simulink subsystem "Subsys_GFolConv_Control"  (R2024b)
settings: Solver=VariableStepAuto  StartTime=0.0  StopTime=10.0  RelTol=1e-3
model mask{S_n=2e6, P_binst=1.5e6, f_n=50, V_n_phph=690, V_n_grid_phph=20e3, V_n_dc=1380, L_filter_conv_pu=[ 0.0001 0.05097 ], C_filter_pu=[ 0.06875 0.04569 ], outputSignal=0, f_sw=5000, send_info_messages=1, T_s_ctrl=1e-4, T_s_PWM_meas=1e-4, datatype='double', meas_signals=0, meas_lowpass=1, meas_f_cutoff_lowpass=2500, meas_f_cutoff_posseq=20, prot_variant=2, v_dc_max=1.2, v_ac_max=1.1, t_ac_max=0.1, v_ac_maxmax=1.25, t_ac_maxmax=0.1, v_ac_min=0.8, t_ac_min=3, v_ac_minmin=0.45, t_ac_minmin=0.3, f_ac_max=51.5, t_f_ac_max=0.1, f_ac_maxmax=52.5, t_f_ac_maxmax=10, f_ac_min=47.5, t_f_ac_min=0.1, i_ac_max=1.25, outer_ctrl_mode=1, VDE4110_T_LPF_P=33e-3, VDE4110_Pf_DBlow=49.8, VDE4110_Pf_DBhigh=50.2, VDE4110_Pf_droop=5, VDE4110_Pf_dPdtmax=1, isStorage=0, Ts_Matching_m=0, K_Matching_m=0, Plant_Ref=0, Plant_Model=0, Luenberger=0, VDE4110_Q_ctrl_mode=3, VDE4110_T_PT1_Q=3.33, VDE4110_QV_uq0ref=1, VDE4110_QV_qmax=0.33, VDE4110_QV_umax=1.04, VDE4110_QV_deadband=0, VDE4110_QP_P=[0.1, 0.5, 0.6, 0.9, 1.0], VDE4110_QP_Q=[0.0, 0.0, -0.05, -0.33, -0.33], VDE4110_QVDB_P1=[0.94, 0.33], VDE4110_QVDB_P2=[0.96, 0], VDE4110_QVDB_P3=[1.04, 0], VDE4110_QVDB_P4=[1.06, -0.33], VDE4110_cosphi_ref=1, VDE4110_cosphi_direction=1, PQ_ctrl_mode=0, K_p_PQ_Ctrl=0.6, K_i_PQ_Ctrl=3.2, K_p_I_Ctrl=0.6, K_i_I_Ctrl=0.6, v_conv_max=1.3, i_grid_max=1.1, active_damping=1, R_virt_pu=0.2}
  mask prompts: S_n "Nominal apparent power [VA]"; P_binst "Installed active power [W]"; f_n "Nominal frequency [Hz]"; V_n_phph "Nominal converter voltage (rms, phase-to-phase) [V]"; V_n_grid_phph "Nominal grid voltage (rms, phase-to-phase) [V]"; V_n_dc "Nominal DC-link voltage [V]"; L_filter_conv_pu "Impedance of converter-side inductance [ R L ] (pu)"; C_filter_pu "Impedance of filter capacitor [ R C ] (pu)"; outputSignal "Output signal type (2 = duty cycle (imperix), 1 = switching pulses, 0 = voltage reference (average model))"; f_sw "Switching frequency [Hz]"; send_info_messages "Send info messages (1 = enabled, 0 = disabled)"; T_s_ctrl "Controller sample time [s]"; T_s_PWM_meas "PWM and measurements sample time [s]"; datatype "Signal data type"; meas_signals "Measured signals (0 = all signals (tDMSquared simulation), 1 = reduced signals (imperix hardware))"; meas_lowpass "Low pass to filter measurement noise (1 = enabled, 0 = disabled)"; meas_f_cutoff_lowpass "Cutoff frequency of low pass filter (measurement noise) [Hz]"; meas_f_cutoff_posseq "Cutoff frequency of low pass filter (positive sequence calculation) [Hz]"; prot_variant "Protection Variant (1= hardware protection, 2 = tDMSquared warnings only, 3 = deactivated)"; v_dc_max "Maximum DC-link voltage [% nom. value]"; v_ac_max "Lower Maximum AC voltage [% nom. value]"; t_ac_max "Lower Maximum AC voltage timing [s]"; v_ac_maxmax "Upper Maximum AC voltage [% nom. value]"; t_ac_maxmax "Upper Maximum AC voltage timing [s]"; v_ac_min "Upper Minimum AC voltage [% nom. value]"; t_ac_min "Upper Minimum AC voltage timing [s]"; v_ac_minmin "Lower Minimum AC voltage [% nom. value]"; t_ac_minmin "Lower Minimum AC voltage timing [s]"; f_ac_max "Maximum AC frequency [Hz]"; t_f_ac_max "Maximum AC frequency timing [s]"; f_ac_maxmax "Upper Maximum AC frequency [Hz]"; t_f_ac_maxmax "Upper Maximum AC frequency timing [s]"; f_ac_min "Minimum AC frequency [Hz]"; t_f_ac_min "Minimum AC frequency timing [s]"; i_ac_max "Maximum AC current [% nom. value]"; outer_ctrl_mode "Outer control mode (1 = VDE 4110, 2 = Matching Control, 3 = no control)"; VDE4110_T_LPF_P "Time constant of active power  PT1 [s]"; VDE4110_Pf_DBlow "P(f) deadband lower limit [Hz]"; VDE4110_Pf_DBhigh "P(f) deadband higher limit [Hz]"; VDE4110_Pf_droop "P(f) droop [(df/f_n)/(dP/Pref)] [%]"; VDE4110_Pf_dPdtmax "P(f) maximum dP/dt [pu / s]"; isStorage "Generation unit is energy storage (1 = true, 0 = false)"; Ts_Matching_m "Time Constant"; K_Matching_m "Feedback Gain"; Plant_Ref "Reference Model"; Plant_Model "Plant Model"; Luenberger "Luenberger Gain"; VDE4110_Q_ctrl_mode "Q-control mode (1 = Q(V), 2 = Q(P), 3 = Q(V) with deadband, 4 = cosphi)"; VDE4110_T_PT1_Q "Time constant of reactive power PT1 delay [s]"; VDE4110_QV_uq0ref "U_Q0ref [pu]"; VDE4110_QV_qmax "|Q_max| [pu]"; VDE4110_QV_umax "U_max [pu]"; VDE4110_QV_deadband "Voltage deadband [+- %]"; VDE4110_QP_P "P_grid points [pu]"; VDE4110_QP_Q "Q_grid points [pu]"; VDE4110_QVDB_P1 "P1 [V_grid, Q_grid] [pu]"; VDE4110_QVDB_P2 "P2 [V_grid, Q_grid] [pu]"; VDE4110_QVDB_P3 "P3 [V_grid, Q_grid] [pu]"; VDE4110_QVDB_P4 "P4 [V_grid, Q_grid] [pu]"; VDE4110_cosphi_ref "cos(phi)"; VDE4110_cosphi_direction "Reactive power flow direction (1 = ind. Q injection, 0 = ind. Q consumption)"; PQ_ctrl_mode "Active/reactive power control mode (closed loop = 0, open loop = 1)"; K_p_PQ_Ctrl "Proportional gain (PI power controller) [pu]"; K_i_PQ_Ctrl "Integral gain (PI power controller) [pu]"; K_p_I_Ctrl "Proportional gain (PI current controller) [pu]"; K_i_I_Ctrl "Integral gain (PI current controller) [pu]"; v_conv_max "Converter voltage maximum value (limit) [pu]"; i_grid_max "Converter current maximum value (limit) [pu]"; active_damping "Active Damping (1 = enabled, 0 = disabled)"; R_virt_pu "Virtual resistor for active damping (in series with converter-side inductance) [pu]"
libraries: simulink x6, eeTransforms x2, eePwmGeneratorTwoLevel x1
settings Model: Creator=winkens  LastModifiedBy=KIVANÇKOCAOĞULLAR
settings SolverCC: AlgebraicLoopSolver=TrustRegion
settings OptimizationCC: ReuseModelBlockBuffer=off
settings DebuggingCC: UnconnectedInputMsg=warning  UnconnectedOutputMsg=warning  UnconnectedLineMsg=warning
settings ModelReferenceCC: EnableRefExpFcnMdlSchedulingChecks=on
settings RTWCC: GPUComputeCapability=3.5  DLArmComputeVersion=19.05

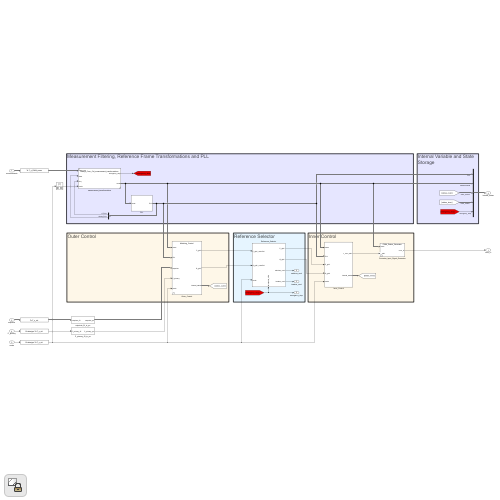
[thumbnail: Simulink's stored preview of the top-level diagram]
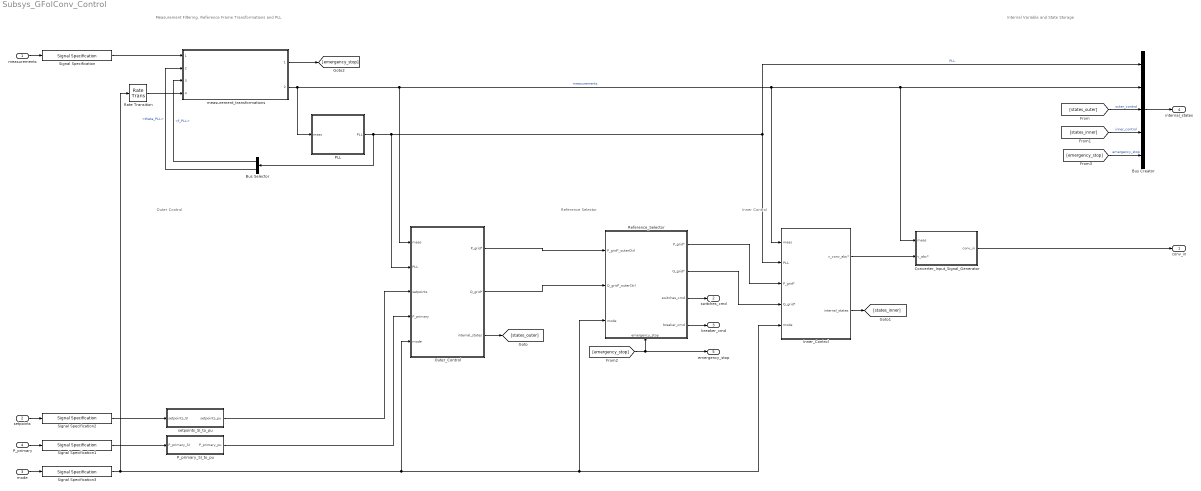
== system Subsys_GFolConv_Control ==
  note: Reference Selector
  note: Measurement Filtering, Reference Frame Transformations and PLL
  note: Outer Control
  note: Inner Control
  note: Internal Variable and State
      | Storage
  measurements : Inport
  setpoints : Inport  Port=2
  mode : Inport  Port=3
  P_primary : Inport  Port=4
  Bus Creator : BusCreator  Inputs=5
  Bus Selector : BusSelector  OutputSignals=f_PLL,theta_PLL
  Converter_Input_Signal_Generator : Subsystem  Variant=on
  Inner_Control : Subsystem
  Outer_Control : Subsystem  Variant=on  VariantControl=Choice
  PLL : Subsystem
  P_primary_SI_to_pu : Subsystem
  Rate Transition : RateTransition  OutPortSampleTime=T_s_PWM_meas
  Reference_Selector : Subsystem
      settings: PortSchema="{\"entries\":[{\"content\":{\"sides\":[{\"content\":{\"connectorIds\":[\"In1\",\"In2\",\"In3\"]},\"type\":\"ConnectorPlacement.EquallySpacedRectSide\",\"uuid\":\"b573c78f-d58c-40ce-b3bc-9375892f1426\"},{\"content\":{\"connectorIds\":[\"Out1\",\"Out2\",\"Out3\",\"Out4\"],\"side\":\"RIGHT\"},\"type\":\"ConnectorPlacement.EquallySpacedRectSide\",\"uuid\":\"e589ace7-4775-4159-9960-f42613345aac\"},{\"content\":{\"connectorIds\":[],\"side\":\"TOP\"},\"type\":\"ConnectorPlacement.EquallySpacedRectSide\",\"uuid\":\"d891a4af-dcc2-49f2-8d70-7d3294665827\"},{\"content\":{\"connectorIds\":[\"In4\"],\"side\":\"BOTTOM\"},\"type\":\"ConnectorPlacement.EquallySpacedRectSide\",\"uuid\":\"20ebcd43-a549-487f-8746-8af8878ad08b\"},{\"content\":{\"connectorIds\":[],\"side\":\"HIDDEN\"},\"type\":\"ConnectorPlacement.EquallySpacedRectSide\",\"uuid\":\"aa9de6de-879f-42fa-ad20-1b3327d10a74\"}]},\"type\":\"ConnectorPlacement.EquallySpacedConnector\",\"uuid\":\"970e3a91-45bd-4cb1-a5f8-11fb4fe15b0f\"}],\"packageUris\":[\"http://schema.mathworks.com/mf0/Connector/R2020b\"],\"version\":\"1.0\"}"
  Signal Specification : SignalSpecification  SampleTime=T_s_PWM_meas
  Signal Specification1 : SignalSpecification  OutDataTypeStr=datatype  SampleTime=T_s_ctrl
  Signal Specification2 : SignalSpecification  SampleTime=T_s_ctrl
  Signal Specification3 : SignalSpecification  OutDataTypeStr=datatype  SampleTime=T_s_ctrl
  measurement_transformations : Subsystem  ReferencedSubsystem=Subsys_Conv_Ctrl_measurement_transformations  S_n=S_n  f_n=f_n  V_n_phph=V_n_phph  V_n_grid_phph=V_n_grid_phph  V_n_dc=V_n_dc  meas_signals=meas_signals  meas_noise_filter=meas_lowpass  f_cutoff_lowpass=meas_f_cutoff_lowpass  posseq_calc=0  f_cutoff_posseq=meas_f_cutoff_posseq  prot_variant=prot_variant  v_dc_max=v_dc_max  v_ac_max=v_ac_max  t_ac_max=t_ac_max  v_ac_maxmax=v_ac_maxmax  t_ac_maxmax=t_ac_maxmax  v_ac_min=v_ac_min  t_ac_min=t_ac_min  v_ac_minmin=v_ac_minmin  t_ac_minmin=t_ac_minmin  f_ac_max=f_ac_max  t_f_ac_max=t_f_ac_max  f_ac_maxmax=f_ac_maxmax  t_f_ac_maxmax=t_f_ac_maxmax  f_ac_min=f_ac_min  t_f_ac_min=t_f_ac_min  i_ac_max=i_ac_max  T_s_ctrl=T_s_ctrl  T_s_PWM_meas=T_s_PWM_meas  datatype=datatype
  setpoints_SI_to_pu : Subsystem
  conv_in : Outport
  switches_cmd : Outport  Port=2
  breaker_cmd : Outport  Port=3
  internal_states : Outport  Port=4
  emergency_stop : Outport  Port=5
  wires:
  Bus Selector/1 -> measurement_transformations/3  "<f_PLL>"
  Reference_Selector/2(Q_grid*) -> Inner_Control/4(Q_grid*)
  Reference_Selector/1(P_grid*) -> Inner_Control/3(P_grid*)
  [emergency_stop] -> Reference_Selector/4(emergency_stop), emergency_stop/1
  Reference_Selector/3(switches_cmd) -> switches_cmd/1
  Reference_Selector/4(breaker_cmd) -> breaker_cmd/1
  Signal Specification2/1 -> setpoints_SI_to_pu/1(setpoints_SI)
  measurement_transformations/1 -> [emergency_stop]
  Bus Selector/2 -> measurement_transformations/2  "<theta_PLL>"
  Signal Specification/1 -> measurement_transformations/1
  Signal Specification3/1 -> Reference_Selector/3(mode), Inner_Control/5(mode), Outer_Control/5(mode), Rate Transition/1
  Signal Specification1/1 -> P_primary_SI_to_pu/1(P_primary_SI)
  P_primary_SI_to_pu/1(P_primary_pu) -> Outer_Control/4(P_primary)
  P_primary/1 -> Signal Specification1/1
  Outer_Control/3(internal_states) -> [states_outer]
  Outer_Control/2(Q_grid*) -> Reference_Selector/2(Q_grid*_outerCtrl)
  Outer_Control/1(P_grid*) -> Reference_Selector/1(P_grid*_outerCtrl)
  setpoints_SI_to_pu/1(setpoints_pu) -> Outer_Control/3(setpoints)
  measurements/1 -> Signal Specification/1
  setpoints/1 -> Signal Specification2/1
  mode/1 -> Signal Specification3/1
  measurement_transformations/2 -> PLL/1(meas), Outer_Control/1(meas), Bus Creator/2, Converter_Input_Signal_Generator/1(meas), Inner_Control/1(meas)  "measurements"
  Inner_Control/1(v_conv_abc*) -> Converter_Input_Signal_Generator/2(v_abc*)
  Inner_Control/2(internal_states) -> [states_inner]
  [states_outer] -> Bus Creator/3  "outer_control"
  [states_inner] -> Bus Creator/4  "inner_control"
  Bus Creator/1 -> internal_states/1
  Converter_Input_Signal_Generator/1(conv_in) -> conv_in/1
  [emergency_stop] -> Bus Creator/5  "emergency_stop"
  Rate Transition/1 -> measurement_transformations/4
  PLL/1(PLL) -> Bus Selector/1, Bus Creator/1, Inner_Control/2(PLL), Outer_Control/2(PLL)  "PLL"

== system Subsys_GFolConv_Control/Converter_Input_Signal_Generator ==
  meas : Inport
  v_abc* : Inport  Port=2
  PWM_Pulses_Generator : Subsystem  VariantControl=outputSignal == 1
  Uref_Signal_Generator : Subsystem  VariantControl=(default)
  imperix_dutycycle_generator : Subsystem  VariantControl=outputSignal == 2
  conv_in : Outport

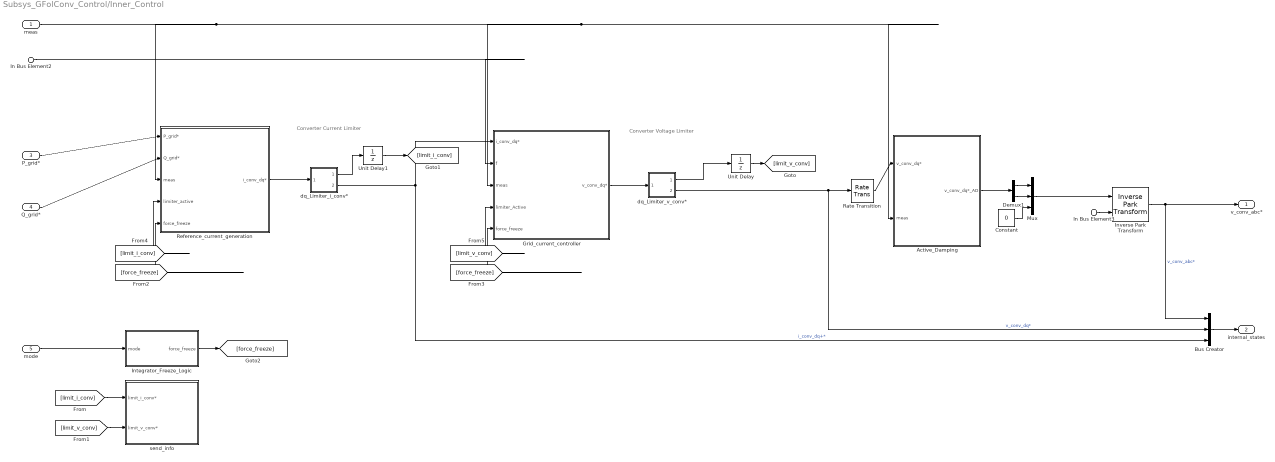
== system Subsys_GFolConv_Control/Inner_Control ==
  note: Converter Current Limiter
  note: Converter Voltage Limiter
  meas : Inport
  In Bus Element2 : Inport  Port=2  PortName=PLL  Element=f_PLL
  In Bus Element3 : Inport  Port=2  PortName=PLL  Element=theta_PLL
  P_grid* : Inport  Port=3
  Q_grid* : Inport  Port=4
  mode : Inport  Port=5
  Active_Damping : Subsystem  Variant=on  VariantControl=Choice
  Bus Creator : BusCreator  Inputs=3
  Constant : Constant  Value=0  OutDataTypeStr=datatype
  Demux1 : Demux  Outputs=2
  Grid_current_controller : Subsystem
  Integrator_Freeze_Logic : Subsystem
  Inverse Park Transform : eeTransforms/Inverse Park Transform  AxisAlignment=D-axis  PowerInvariant=off
  Mux : Mux  Inputs=3
  Rate Transition : RateTransition  Deterministic=off  OutPortSampleTime=T_s_PWM_meas
  Reference_current_generation : Subsystem  Variant=on  VariantControl=Choice
  Unit Delay : UnitDelay  SampleTime=-1  HasFrameUpgradeWarning=on
  Unit Delay1 : UnitDelay  SampleTime=-1  HasFrameUpgradeWarning=on
  dq_Limiter_i_conv* : Subsystem  ReferencedSubsystem=dq_Limiter  X_dq_max=i_grid_max  datatype=datatype
  dq_Limiter_v_conv* : Subsystem  ReferencedSubsystem=dq_Limiter  X_dq_max=v_conv_max  datatype=datatype
  send_info : Subsystem  Variant=on
  v_conv_abc* : Outport
  internal_states : Outport  Port=2
  wires:
  Integrator_Freeze_Logic/1(force_freeze) -> [force_freeze]
  mode/1 -> Integrator_Freeze_Logic/1(mode)
  Unit Delay1/1 -> [limit_i_conv]
  Reference_current_generation/1(i_conv_dq*) -> dq_Limiter_i_conv*/1
  dq_Limiter_i_conv*/1 -> Unit Delay1/1
  P_grid*/1 -> Reference_current_generation/1(P_grid*)
  Q_grid*/1 -> Reference_current_generation/2(Q_grid*)
  dq_Limiter_v_conv*/1 -> Unit Delay/1
  dq_Limiter_v_conv*/2 -> Bus Creator/2, Rate Transition/1  "v_conv_dq*"
  Unit Delay/1 -> [limit_v_conv]
  Mux/1 -> Inverse Park Transform/1
  Constant/1 -> Mux/3
  Demux1/2 -> Mux/2
  Demux1/1 -> Mux/1
  meas/1 -> Grid_current_controller/3(meas), Active_Damping/2(meas), Reference_current_generation/3(meas)
  In Bus Element2/1 -> Grid_current_controller/2(f)
  In Bus Element3/1 -> Inverse Park Transform/2
  Inverse Park Transform/1 -> Bus Creator/1, v_conv_abc*/1  "v_conv_abc*"
  Bus Creator/1 -> internal_states/1
  dq_Limiter_i_conv*/2 -> Bus Creator/3, Grid_current_controller/1(i_conv_dq*)  "i_conv_dq+*"
  Grid_current_controller/1(v_conv_dq*) -> dq_Limiter_v_conv*/1
  Rate Transition/1 -> Active_Damping/1(v_conv_dq*)
  Active_Damping/1(v_conv_dq*_AD) -> Demux1/1
  [limit_i_conv] -> send_info/1(limit_i_conv*)
  [limit_v_conv] -> send_info/2(limit_v_conv*)
  [force_freeze] -> Reference_current_generation/5(force_freeze)
  [force_freeze] -> Grid_current_controller/5(force_freeze)
  [limit_i_conv] -> Reference_current_generation/4(limiter_active)
  [limit_v_conv] -> Grid_current_controller/4(limiter_Active)

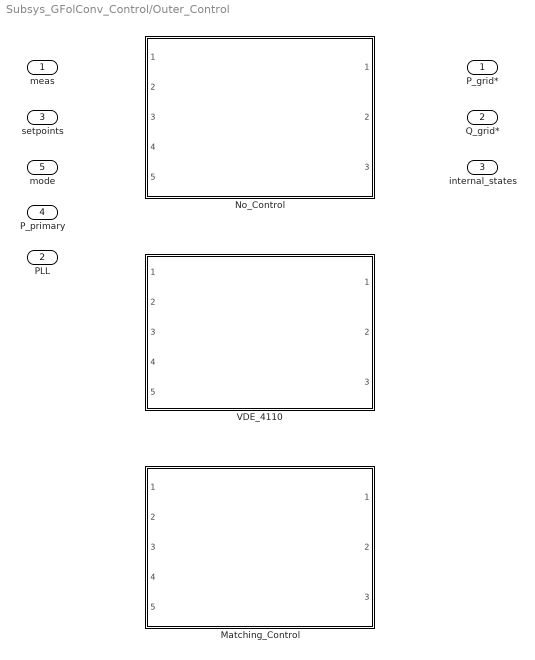
== system Subsys_GFolConv_Control/Outer_Control ==
  meas : Inport
  PLL : Inport  Port=2
  setpoints : Inport  Port=3
  P_primary : Inport  Port=4
  mode : Inport  Port=5
  Matching_Control : Subsystem  VariantControl=outer_ctrl_mode == 2  ReferencedSubsystem=Subsys_GFolConv_OuterCtrl_MatchCtrl  S_n=S_n  P_binst=P_binst  f_n=f_n  Q_ctrl_mode_m=VDE4110_Q_ctrl_mode  T_PT1_Q_m=VDE4110_T_PT1_Q  uq0ref_m=VDE4110_QV_uq0ref  qmax_m=VDE4110_QV_qmax  umax_m=VDE4110_QV_umax  deadband_m=VDE4110_QV_deadband  p_pu_m=VDE4110_QP_P  q_pu_m=VDE4110_QP_Q  p1_m=VDE4110_QVDB_P1  p2_m=VDE4110_QVDB_P2  p3_m=VDE4110_QVDB_P3  p4_m=VDE4110_QVDB_P4  cosphi_ref_m=VDE4110_cosphi_ref  Q_direction_m=VDE4110_cosphi_direction  T_s_ctrl=T_s_ctrl  datatype=datatype  K_matching=K_Matching_m  plant_ref=Plant_Ref  plant_model=Plant_Model  luenberger=Luenberger  Ts_matching=Ts_Matching_m
  No_Control : Subsystem  VariantControl=outer_ctrl_mode == 3  ReferencedSubsystem=Subsys_GFolConv_OuterCtrl_NoCtrl  T_s_ctrl=T_s_ctrl  datatype=datatype
  VDE_4110 : Subsystem  VariantControl=(default)  ReferencedSubsystem=Subsys_GFolConv_OuterCtrl_VDE4110  S_n=S_n  P_binst=P_binst  f_n=f_n  T_LPF_P=VDE4110_T_LPF_P  VDE4110_Pf_DBlow=VDE4110_Pf_DBlow  VDE4110_Pf_DBhigh=VDE4110_Pf_DBhigh  VDE4110_Pf_droop=VDE4110_Pf_droop  VDE4110_Pf_dPdt_max=VDE4110_Pf_dPdtmax  VDE4110_Pf_isStorage=isStorage  Q_ctrl_mode=VDE4110_Q_ctrl_mode  T_PT1_Q=VDE4110_T_PT1_Q  uq0ref=VDE4110_QV_uq0ref  qmax=VDE4110_QV_qmax  umax=VDE4110_QV_umax  deadband=VDE4110_QV_deadband  p_pu=VDE4110_QP_P  q_pu=VDE4110_QP_Q  p1=VDE4110_QVDB_P1  p2=VDE4110_QVDB_P2  p3=VDE4110_QVDB_P3  p4=VDE4110_QVDB_P4  cosphi_ref=VDE4110_cosphi_ref  Q_direction=VDE4110_cosphi_direction  T_s_ctrl=T_s_ctrl  datatype=datatype
  P_grid* : Outport
  Q_grid* : Outport  Port=2
  internal_states : Outport  Port=3

== system Subsys_GFolConv_Control/PLL ==
  In Bus Element : Inport  PortName=meas  Element=dq+.v_cap_dq+
  Gain : Gain  Gain=1/f_n
  Rate Transition1 : RateTransition  Deterministic=off  OutPortSampleTime=T_s_ctrl
  Rate Transition2 : RateTransition  Deterministic=off  OutPortSampleTime=T_s_PWM_meas
  Signal Specification : SignalSpecification  OutDataTypeStr=datatype  SampleTime=T_s_PWM_meas
  Signal Specification1 : SignalSpecification  OutDataTypeStr=datatype  SampleTime=T_s_PWM_meas
  Subsystem Reference : Subsystem  ReferencedSubsystem=PLL  f_n=f_n  K_p=25.13  K_i=15791  df_max=f_n  f_c=25  theta_feedback=0  T_s=T_s_PWM_meas  datatype=datatype
  Bus Element Out : Outport  PortName=PLL  Element=theta_PLL
  Out Bus Element : Outport  PortName=PLL  Element=f_PLL
  wires:
  Rate Transition1/1 -> Out Bus Element/1
  In Bus Element/1 -> Rate Transition2/1
  Subsystem Reference/2 -> Signal Specification1/1
  Signal Specification/1 -> Gain/1
  Subsystem Reference/1 -> Signal Specification/1
  Gain/1 -> Rate Transition1/1
  Rate Transition2/1 -> Subsystem Reference/1
  Signal Specification1/1 -> Bus Element Out/1

== system Subsys_GFolConv_Control/P_primary_SI_to_pu ==
  P_primary_SI : Inport
  Gain : Gain  Gain=1/S_n
  P_primary_pu : Outport
  wires:
  Gain/1 -> P_primary_pu/1
  P_primary_SI/1 -> Gain/1

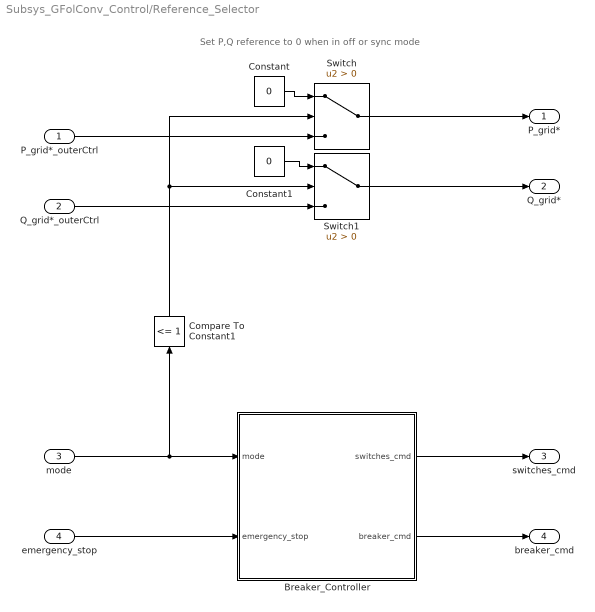
== system Subsys_GFolConv_Control/Reference_Selector ==
  note: Set P,Q reference to 0 when in off or sync mode
  P_grid*_outerCtrl : Inport
  Q_grid*_outerCtrl : Inport  Port=2
  mode : Inport  Port=3
  emergency_stop : Inport  Port=4
  Breaker_Controller : Subsystem
  Compare To Constant1 : simulink/Logic and Bit Operations/Compare To Constant  relop=<=  const=1  OutDataTypeStr=boolean
  Constant : Constant  Value=0  OutDataTypeStr=datatype
  Constant1 : Constant  Value=0  OutDataTypeStr=datatype
  Switch : Switch  Criteria=u2 > Threshold  SaturateOnIntegerOverflow=off  InputSameDT=off
  Switch1 : Switch  Criteria=u2 > Threshold  SaturateOnIntegerOverflow=off  InputSameDT=off
  P_grid* : Outport
  Q_grid* : Outport  Port=2
  switches_cmd : Outport  Port=3
  breaker_cmd : Outport  Port=4
  wires:
  Switch1/1 -> Q_grid*/1
  Switch/1 -> P_grid*/1
  P_grid*_outerCtrl/1 -> Switch/3
  Constant1/1 -> Switch1/1
  Constant/1 -> Switch/1
  Compare To Constant1/1 -> Switch/2, Switch1/2
  Q_grid*_outerCtrl/1 -> Switch1/3
  mode/1 -> Breaker_Controller/1(mode), Compare To Constant1/1
  emergency_stop/1 -> Breaker_Controller/2(emergency_stop)
  Breaker_Controller/1(switches_cmd) -> switches_cmd/1
  Breaker_Controller/2(breaker_cmd) -> breaker_cmd/1

== system Subsys_GFolConv_Control/setpoints_SI_to_pu ==
  Bus Element In : Inport  PortName=setpoints_SI  Element=P_set
  In Bus Element : Inport  PortName=setpoints_SI  Element=Q_set
  Bus Creator : BusCreator  Inputs=2
  Gain : Gain  Gain=1/S_n
  Gain1 : Gain  Gain=1/S_n
  setpoints_pu : Outport
  wires:
  Bus Creator/1 -> setpoints_pu/1
  Gain1/1 -> Bus Creator/2  "Q_set_pu"
  Gain/1 -> Bus Creator/1  "P_set_pu"
  In Bus Element/1 -> Gain1/1
  Bus Element In/1 -> Gain/1

== system Subsys_GFolConv_Control/Converter_Input_Signal_Generator/PWM_Pulses_Generator ==
  Bus Element In : Inport  PortName=meas  Element=v_dc
  v_abc* : Inport  Port=2
  Gain : Gain  Gain=V_n_dc*sqrt(3/2)/V_n_phph
  PWM_Generator : eePwmGeneratorTwoLevel/PWM Generator (Three-phase, Two-level)  PWMMode=Continuous PWM (CPWM)  CPWMMode=SPWM: sinusoidal PWM  DPWMMode=60 DPWM: 60 degree discontinuous PWM  fsw=f_sw  Ts=T_s_PWM_meas(1)
  Terminator : Terminator
  conv_in : Outport
  wires:
  Bus Element In/1 -> Gain/1
  v_abc*/1 -> PWM_Generator/1
  PWM_Generator/1 -> conv_in/1
  PWM_Generator/2 -> Terminator/1
  Gain/1 -> PWM_Generator/2

== system Subsys_GFolConv_Control/Converter_Input_Signal_Generator/Uref_Signal_Generator ==
  Bus Element In : Inport  PortName=meas  Element=v_dc
  v_abc* : Inport  Port=2
  Constant : Constant  Value=2  OutDataTypeStr=datatype
  Demux : Demux  Outputs=3
  Divide : Product  Inputs=**/
  Gain : Gain  Gain=V_n_dc*sqrt(3/2)/V_n_phph
  Ground : Ground
  Mux : Mux  Inputs=6
  conv_in : Outport
  wires:
  v_abc*/1 -> Divide/1
  Bus Element In/1 -> Gain/1
  Constant/1 -> Divide/2
  Demux/1 -> Mux/1
  Demux/2 -> Mux/2
  Demux/3 -> Mux/3
  Ground/1 -> Mux/6, Mux/4, Mux/5
  Mux/1 -> conv_in/1
  Divide/1 -> Demux/1
  Gain/1 -> Divide/3

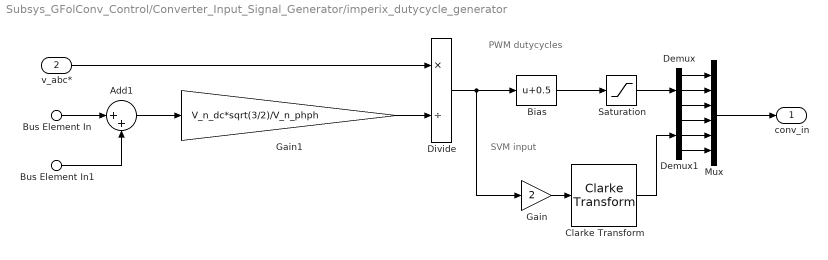
== system Subsys_GFolConv_Control/Converter_Input_Signal_Generator/imperix_dutycycle_generator ==
  note: SVM input
  note: PWM dutycycles
  Bus Element In : Inport  PortName=meas  Element=v_dc_low
  Bus Element In1 : Inport  PortName=meas  Element=v_dc_up
  v_abc* : Inport  Port=2
  Add1 : Sum  Inputs=|++
  Bias : Bias  Bias=0.5  SaturateOnIntegerOverflow=off
  Clarke Transform : eeTransforms/Clarke Transform  PowerInvariant=off
  Demux : Demux  Outputs=3
  Demux1 : Demux  Outputs=3
  Divide : Product  Inputs=*/
  Gain : Gain  Gain=2
  Gain1 : Gain  Gain=V_n_dc*sqrt(3/2)/V_n_phph
  Mux : Mux  Inputs=6
  Saturation : Saturate  UpperLimit=1  LowerLimit=0
  conv_in : Outport
  wires:
  Saturation/1 -> Demux/1
  v_abc*/1 -> Divide/1
  Bus Element In1/1 -> Add1/2
  Bias/1 -> Saturation/1
  Mux/1 -> conv_in/1
  Divide/1 -> Bias/1, Gain/1
  Demux/1 -> Mux/1
  Bus Element In/1 -> Add1/1
  Demux/3 -> Mux/3
  Demux/2 -> Mux/2
  Clarke Transform/1 -> Demux1/1
  Demux1/3 -> Mux/6
  Demux1/2 -> Mux/5
  Demux1/1 -> Mux/4
  Gain/1 -> Clarke Transform/1
  Add1/1 -> Gain1/1
  Gain1/1 -> Divide/2

== system Subsys_GFolConv_Control/Inner_Control/Active_Damping ==
  v_conv_dq* : Inport
  meas : Inport  Port=2
  No_Damping : Subsystem  VariantControl=(default)
  Virtual_Resistor : Subsystem  VariantControl=active_damping > 0.5
  v_conv_dq*_AD : Outport

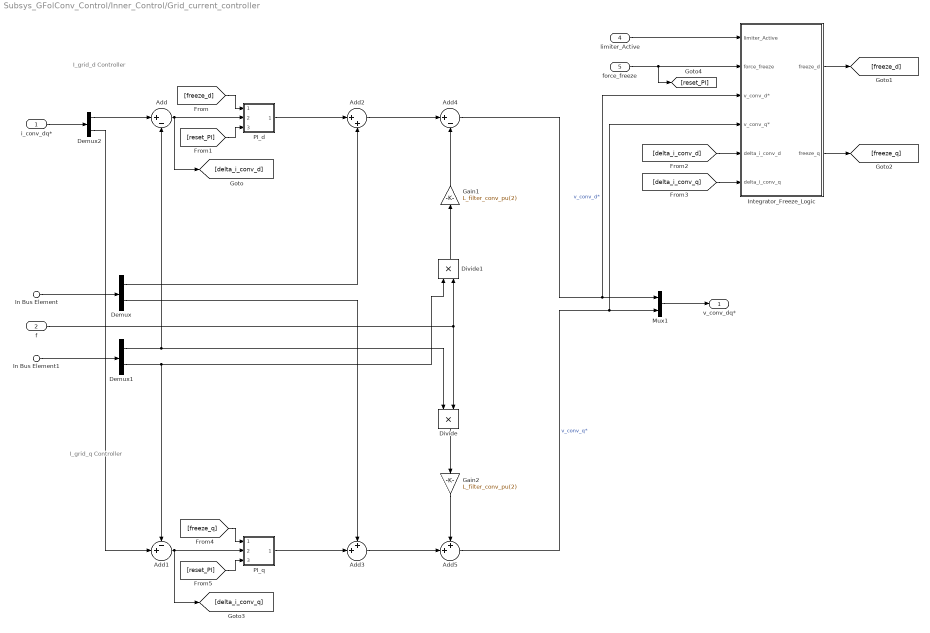
== system Subsys_GFolConv_Control/Inner_Control/Grid_current_controller ==
  note: I_grid_q Controller
  note: I_grid_d Controller
  i_conv_dq* : Inport
  f : Inport  Port=2
  In Bus Element : Inport  Port=3  PortName=meas  Element=dq+.v_cap_dq+
  In Bus Element1 : Inport  Port=3  PortName=meas  Element=dq+.i_conv_dq+
  limiter_Active : Inport  Port=4
  force_freeze : Inport  Port=5
  Add : Sum  Inputs=|+-
  Add1 : Sum  Inputs=-+|
  Add2 : Sum  Inputs=|++
  Add3 : Sum  Inputs=++|
  Add4 : Sum  Inputs=|+-
  Add5 : Sum  Inputs=++|
  Demux : Demux  Outputs=2
  Demux1 : Demux  Outputs=2
  Demux2 : Demux  Outputs=2
  Divide : Product  Inputs=**
  Divide1 : Product  Inputs=**
  Gain1 : Gain  Gain=L_filter_conv_pu(2)
  Gain2 : Gain  Gain=L_filter_conv_pu(2)
  Integrator_Freeze_Logic : Subsystem
  Mux1 : Mux  Inputs=2
  PI_d : Subsystem  ReferencedSubsystem=PI_freeze  K_p=K_p_I_Ctrl  K_i=K_i_I_Ctrl  T_s=T_s_ctrl  datatype=datatype
  PI_q : Subsystem  ReferencedSubsystem=PI_freeze  K_p=K_p_I_Ctrl  K_i=K_i_I_Ctrl  T_s=T_s_ctrl  datatype=datatype
  v_conv_dq* : Outport
  wires:
  Demux2/1 -> Add/1
  Demux/1 -> Add2/2
  In Bus Element/1 -> Demux/1
  In Bus Element1/1 -> Demux1/1
  i_conv_dq*/1 -> Demux2/1
  Demux1/1 -> Add/2, Divide/1
  Demux2/2 -> Add1/2
  Demux1/2 -> Add1/1, Divide1/1
  Add/1 -> [delta_i_conv_d], PI_d/2
  Add1/1 -> [delta_i_conv_q], PI_q/2
  PI_d/1 -> Add2/1
  PI_q/1 -> Add3/2
  Add2/1 -> Add4/1
  Add3/1 -> Add5/2
  Demux/2 -> Add3/1
  Divide/1 -> Gain2/1
  Divide1/1 -> Gain1/1
  f/1 -> Divide/2, Divide1/2
  Gain1/1 -> Add4/2
  Gain2/1 -> Add5/1
  Mux1/1 -> v_conv_dq*/1
  limiter_Active/1 -> Integrator_Freeze_Logic/1(limiter_Active)
  [delta_i_conv_d] -> Integrator_Freeze_Logic/5(delta_i_conv_d)
  [delta_i_conv_q] -> Integrator_Freeze_Logic/6(delta_i_conv_q)
  force_freeze/1 -> Integrator_Freeze_Logic/2(force_freeze), [reset_PI]
  Integrator_Freeze_Logic/2(freeze_q) -> [freeze_q]
  Integrator_Freeze_Logic/1(freeze_d) -> [freeze_d]
  Add5/1 -> Integrator_Freeze_Logic/4(v_conv_q*), Mux1/2  "v_conv_q*"
  Add4/1 -> Integrator_Freeze_Logic/3(v_conv_d*), Mux1/1  "v_conv_d*"
  [freeze_d] -> PI_d/1
  [reset_PI] -> PI_d/3
  [freeze_q] -> PI_q/1
  [reset_PI] -> PI_q/3

== system Subsys_GFolConv_Control/Inner_Control/Integrator_Freeze_Logic ==
  note: Freeze Integrators of Inner Control when Converter is deactivated (Modes -1 and 1)
  mode : Inport
  Constant : Constant  OutDataTypeStr=boolean
  Constant3 : Constant  OutDataTypeStr=boolean
  Constant4 : Constant  OutDataTypeStr=boolean
  Constant5 : Constant  Value=0  OutDataTypeStr=boolean
  Multiport Switch2 : MultiPortSwitch  DataPortOrder=Specify indices  DataPortIndices={-1,0,1,[2,3]}  SaturateOnIntegerOverflow=off  InputSameDT=off
  force_freeze : Outport
  wires:
  Constant5/1 -> Multiport Switch2/5
  Constant4/1 -> Multiport Switch2/3
  Constant3/1 -> Multiport Switch2/4
  Constant/1 -> Multiport Switch2/2
  mode/1 -> Multiport Switch2/1
  Multiport Switch2/1 -> force_freeze/1  "force_freeze"

== system Subsys_GFolConv_Control/Inner_Control/Reference_current_generation ==
  P_grid* : Inport
  Q_grid* : Inport  Port=2
  meas : Inport  Port=3
  limiter_active : Inport  Port=4
  force_freeze : Inport  Port=5
  Closed_loop_PQ_control : Subsystem  VariantControl=(default)
  Open_loop_PQ_control : Subsystem  VariantControl=PQ_ctrl_mode == 1
  i_conv_dq* : Outport

== system Subsys_GFolConv_Control/Inner_Control/send_info ==
  limit_i_conv* : Inport
  limit_v_conv* : Inport  Port=2
  no_message : Subsystem  VariantControl=(default)
  send_info : Subsystem  VariantControl=send_info_messages > 0.5

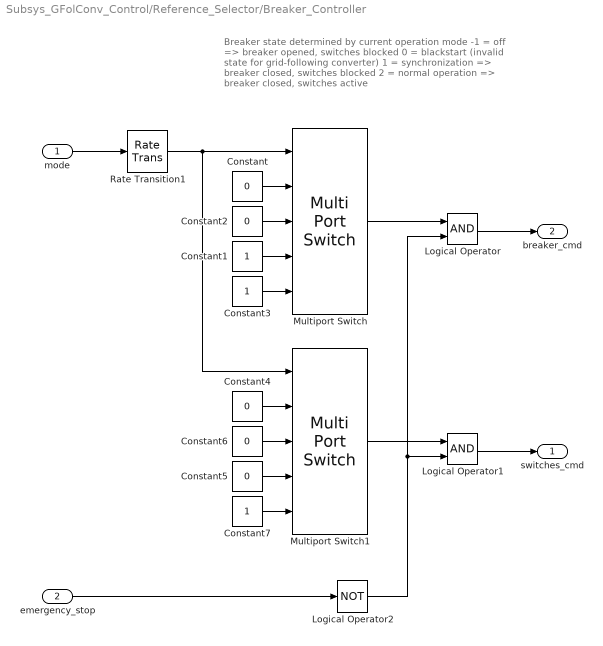
== system Subsys_GFolConv_Control/Reference_Selector/Breaker_Controller ==
  note: Breaker state determined by current operation mode
      | -1 = off => breaker opened, switches blocked
      | 0  = blackstart (invalid state for grid-following converter)
      | 1  = synchronization => breaker closed, switches blocked
      | 2  = normal operation => breaker closed, switches active
  mode : Inport
  emergency_stop : Inport  Port=2
  Constant{,2,4..6} (5 alike) : Constant  Value=0  OutDataTypeStr=boolean
  Constant1 : Constant  OutDataTypeStr=boolean
  Constant3 : Constant  OutDataTypeStr=boolean
  Constant7 : Constant  OutDataTypeStr=boolean
  Logical Operator : Logic  AllPortsSameDT=off  OutDataTypeStr=boolean
  Logical Operator1 : Logic  AllPortsSameDT=off  OutDataTypeStr=boolean
  Logical Operator2 : Logic  Operator=NOT  AllPortsSameDT=off  OutDataTypeStr=boolean
  Multiport Switch : MultiPortSwitch  DataPortOrder=Specify indices  DataPortIndices={-1,0,1,[2,3]}  SaturateOnIntegerOverflow=off  InputSameDT=off
  Multiport Switch1 : MultiPortSwitch  DataPortOrder=Specify indices  DataPortIndices={-1,0,1,[2,3]}  SaturateOnIntegerOverflow=off  InputSameDT=off
  Rate Transition1 : RateTransition  Deterministic=off  OutPortSampleTime=T_s_PWM_meas
  switches_cmd : Outport
  breaker_cmd : Outport  Port=2
  wires:
  Rate Transition1/1 -> Multiport Switch1/1, Multiport Switch/1
  Logical Operator2/1 -> Logical Operator1/2, Logical Operator/2
  emergency_stop/1 -> Logical Operator2/1
  Logical Operator/1 -> breaker_cmd/1
  Logical Operator1/1 -> switches_cmd/1
  mode/1 -> Rate Transition1/1
  Multiport Switch/1 -> Logical Operator/1
  Constant/1 -> Multiport Switch/2
  Constant1/1 -> Multiport Switch/4
  Constant2/1 -> Multiport Switch/3
  Constant3/1 -> Multiport Switch/5
  Multiport Switch1/1 -> Logical Operator1/1
  Constant6/1 -> Multiport Switch1/3
  Constant7/1 -> Multiport Switch1/5
  Constant5/1 -> Multiport Switch1/4
  Constant4/1 -> Multiport Switch1/2

== system Subsys_GFolConv_Control/Inner_Control/Active_Damping/No_Damping ==
  meas : Inport
  v_conv_dq* : Inport  Port=2
  Terminator : Terminator
  v_conv_dq*_AD : Outport
  wires:
  meas/1 -> Terminator/1
  v_conv_dq*/1 -> v_conv_dq*_AD/1

== system Subsys_GFolConv_Control/Inner_Control/Active_Damping/Virtual_Resistor ==
  Bus Element In : Inport  PortName=meas  Element=dq0.i_conv_dq0
  v_conv_dq* : Inport  Port=2
  AD Resistor : Gain  Gain=R_virt_pu
  Add : Sum  Inputs=-+|
  Selector : Selector  InputPortWidth=3  IndexOptions=Index vector (dialog)  Indices=[1 2]  OutputSizes=1
  v_conv_dq*_AD : Outport
  wires:
  AD Resistor/1 -> Add/1
  Add/1 -> v_conv_dq*_AD/1
  v_conv_dq*/1 -> Add/2
  Selector/1 -> AD Resistor/1
  Bus Element In/1 -> Selector/1

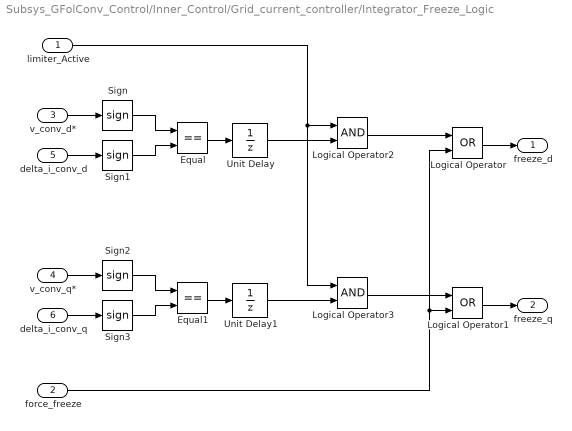
== system Subsys_GFolConv_Control/Inner_Control/Grid_current_controller/Integrator_Freeze_Logic ==
  limiter_Active : Inport
  force_freeze : Inport  Port=2
  v_conv_d* : Inport  Port=3
  v_conv_q* : Inport  Port=4
  delta_i_conv_d : Inport  Port=5
  delta_i_conv_q : Inport  Port=6
  Equal : RelationalOperator  Operator===  OutDataTypeStr=boolean  RndMeth=Simplest  InputSameDT=off
  Equal1 : RelationalOperator  Operator===  OutDataTypeStr=boolean  RndMeth=Simplest  InputSameDT=off
  Logical Operator : Logic  Operator=OR  AllPortsSameDT=off  OutDataTypeStr=boolean
  Logical Operator1 : Logic  Operator=OR  AllPortsSameDT=off  OutDataTypeStr=boolean
  Logical Operator2 : Logic  AllPortsSameDT=off  OutDataTypeStr=boolean
  Logical Operator3 : Logic  AllPortsSameDT=off  OutDataTypeStr=boolean
  Sign{,1..3} (4 alike) : Signum
  Unit Delay : UnitDelay  SampleTime=-1  HasFrameUpgradeWarning=on
  Unit Delay1 : UnitDelay  SampleTime=-1  HasFrameUpgradeWarning=on
  freeze_d : Outport
  freeze_q : Outport  Port=2
  wires:
  Unit Delay1/1 -> Logical Operator3/2
  Unit Delay/1 -> Logical Operator2/2
  v_conv_q*/1 -> Sign2/1
  delta_i_conv_q/1 -> Sign3/1
  Sign2/1 -> Equal1/1
  Sign3/1 -> Equal1/2
  Equal1/1 -> Unit Delay1/1
  Equal/1 -> Unit Delay/1
  Sign1/1 -> Equal/2
  Sign/1 -> Equal/1
  delta_i_conv_d/1 -> Sign1/1
  v_conv_d*/1 -> Sign/1
  Logical Operator3/1 -> Logical Operator1/1
  Logical Operator2/1 -> Logical Operator/1
  limiter_Active/1 -> Logical Operator2/1, Logical Operator3/1
  force_freeze/1 -> Logical Operator1/2, Logical Operator/2
  Logical Operator1/1 -> freeze_q/1
  Logical Operator/1 -> freeze_d/1

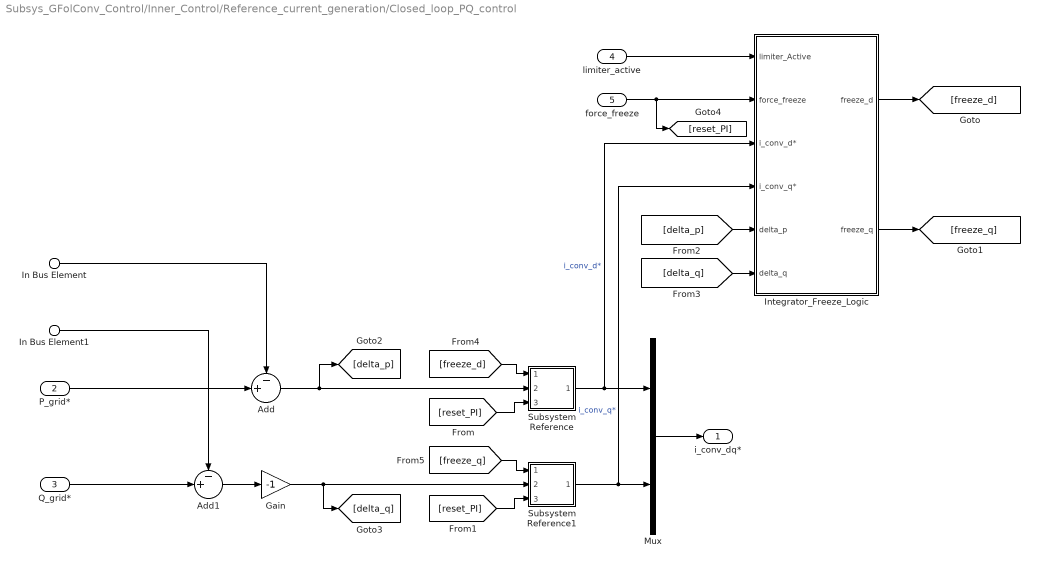
== system Subsys_GFolConv_Control/Inner_Control/Reference_current_generation/Closed_loop_PQ_control ==
  In Bus Element : Inport  PortName=meas  Element=p_grid
  In Bus Element1 : Inport  PortName=meas  Element=q_grid
  P_grid* : Inport  Port=2
  Q_grid* : Inport  Port=3
  limiter_active : Inport  Port=4
  force_freeze : Inport  Port=5
  Add : Sum  Inputs=-+|
  Add1 : Sum  Inputs=-+|
  Gain : Gain  Gain=-1
  Integrator_Freeze_Logic : Subsystem
  Mux : Mux  Inputs=2
  Subsystem Reference : Subsystem  ReferencedSubsystem=PI_freeze  K_p=K_p_PQ_Ctrl  K_i=K_i_PQ_Ctrl  T_s=T_s_ctrl  datatype=datatype
  Subsystem Reference1 : Subsystem  ReferencedSubsystem=PI_freeze  K_p=K_p_PQ_Ctrl  K_i=K_i_PQ_Ctrl  T_s=T_s_ctrl  datatype=datatype
  i_conv_dq* : Outport
  wires:
  Gain/1 -> [delta_q], Subsystem Reference1/2
  Add1/1 -> Gain/1
  Add/1 -> [delta_p], Subsystem Reference/2
  In Bus Element1/1 -> Add1/1
  In Bus Element/1 -> Add/1
  Q_grid*/1 -> Add1/2
  P_grid*/1 -> Add/2
  Mux/1 -> i_conv_dq*/1
  [delta_q] -> Integrator_Freeze_Logic/6(delta_q)
  force_freeze/1 -> Integrator_Freeze_Logic/2(force_freeze), [reset_PI]
  Integrator_Freeze_Logic/1(freeze_d) -> [freeze_d]
  Integrator_Freeze_Logic/2(freeze_q) -> [freeze_q]
  [delta_p] -> Integrator_Freeze_Logic/5(delta_p)
  limiter_active/1 -> Integrator_Freeze_Logic/1(limiter_Active)
  Subsystem Reference/1 -> Integrator_Freeze_Logic/3(i_conv_d*), Mux/1  "i_conv_d*"
  Subsystem Reference1/1 -> Integrator_Freeze_Logic/4(i_conv_q*), Mux/2  "i_conv_q*"
  [reset_PI] -> Subsystem Reference/3
  [reset_PI] -> Subsystem Reference1/3
  [freeze_d] -> Subsystem Reference/1
  [freeze_q] -> Subsystem Reference1/1

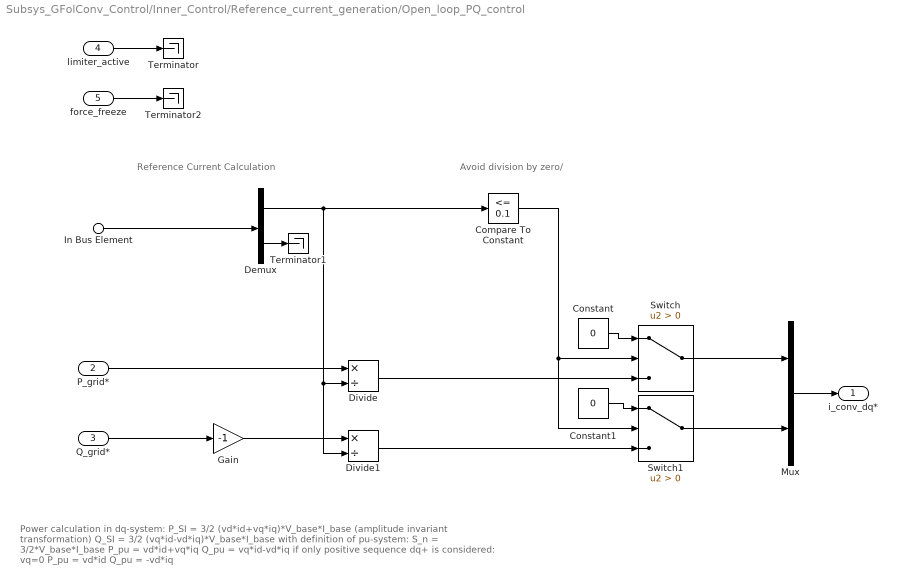
== system Subsys_GFolConv_Control/Inner_Control/Reference_current_generation/Open_loop_PQ_control ==
  note: Avoid division by zero/
  note: Reference Current Calculation
  note: Power calculation in dq-system:
      | P_SI = 3/2 (vd*id+vq*iq)*V_base*I_base (amplitude invariant transformation)
      | Q_SI = 3/2 (vq*id-vd*iq)*V_base*I_base
      | with definition of pu-system: S_n = 3/2*V_base*I_base
      | P_pu = vd*id+vq*iq
      | Q_pu = vq*id-vd*iq
      | if only positive sequence dq+ is considered: vq=0
      | P_pu = vd*id
      | Q_pu = -vd*iq
  In Bus Element : Inport  PortName=meas  Element=dq+.v_cap_dq+
  P_grid* : Inport  Port=2
  Q_grid* : Inport  Port=3
  limiter_active : Inport  Port=4
  force_freeze : Inport  Port=5
  Compare To Constant : simulink/Logic and Bit Operations/Compare To Constant  relop=<=  const=0.1  OutDataTypeStr=boolean
  Constant : Constant  Value=0  OutDataTypeStr=datatype
  Constant1 : Constant  Value=0  OutDataTypeStr=datatype
  Demux : Demux  Outputs=2
  Divide : Product  Inputs=*/
  Divide1 : Product  Inputs=*/
  Gain : Gain  Gain=-1
  Mux : Mux  Inputs=2
  Switch : Switch  Criteria=u2 > Threshold  SaturateOnIntegerOverflow=off  InputSameDT=off
  Switch1 : Switch  Criteria=u2 > Threshold  SaturateOnIntegerOverflow=off  InputSameDT=off
  Terminator : Terminator
  Terminator1 : Terminator
  Terminator2 : Terminator
  i_conv_dq* : Outport
  wires:
  In Bus Element/1 -> Demux/1
  Q_grid*/1 -> Gain/1
  P_grid*/1 -> Divide/1
  Gain/1 -> Divide1/1
  Demux/1 -> Divide/2, Divide1/2, Compare To Constant/1
  Demux/2 -> Terminator1/1
  Mux/1 -> i_conv_dq*/1
  Divide/1 -> Switch/3
  Divide1/1 -> Switch1/3
  Switch/1 -> Mux/1
  Switch1/1 -> Mux/2
  Constant/1 -> Switch/1
  Constant1/1 -> Switch1/1
  Compare To Constant/1 -> Switch/2, Switch1/2
  force_freeze/1 -> Terminator2/1
  limiter_active/1 -> Terminator/1

== system Subsys_GFolConv_Control/Inner_Control/send_info/no_message ==
  limit_i_conv* : Inport
  limit_v_conv* : Inport  Port=2
  Terminator : Terminator
  Terminator1 : Terminator
  wires:
  limit_v_conv*/1 -> Terminator1/1
  limit_i_conv*/1 -> Terminator/1

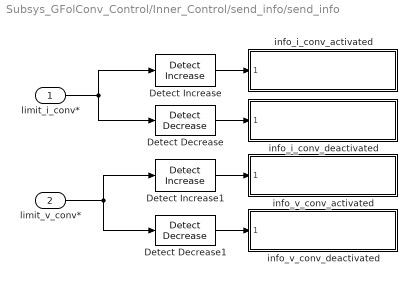
== system Subsys_GFolConv_Control/Inner_Control/send_info/send_info ==
  limit_i_conv* : Inport
  limit_v_conv* : Inport  Port=2
  Detect Decrease : simulink/Logic and Bit Operations/Detect Decrease  vinit=0.0  OutDataTypeStr=boolean
  Detect Decrease1 : simulink/Logic and Bit Operations/Detect Decrease  vinit=0.0  OutDataTypeStr=boolean
  Detect Increase : simulink/Logic and Bit Operations/Detect Increase  vinit=0.0  OutDataTypeStr=boolean
  Detect Increase1 : simulink/Logic and Bit Operations/Detect Increase  vinit=0.0  OutDataTypeStr=boolean
  info_i_conv_activated : Subsystem  ReferencedSubsystem=tDMSquared_Info  messageText='The converter current setpoint (i_conv*) limiter is activated.'  T_s=T_s_ctrl
  info_i_conv_deactivated : Subsystem  ReferencedSubsystem=tDMSquared_Info  messageText='The converter current setpoint (i_conv*) limiter is deactivated.'  T_s=T_s_ctrl
  info_v_conv_activated : Subsystem  ReferencedSubsystem=tDMSquared_Info  messageText='The converter voltage setpoint (v_conv*) limiter is activated.'  T_s=T_s_ctrl
  info_v_conv_deactivated : Subsystem  ReferencedSubsystem=tDMSquared_Info  messageText='The converter voltage setpoint (v_conv*) limiter is deactivated.'  T_s=T_s_ctrl
  wires:
  Detect Increase/1 -> info_i_conv_activated/1
  Detect Decrease/1 -> info_i_conv_deactivated/1
  Detect Decrease1/1 -> info_v_conv_deactivated/1
  Detect Increase1/1 -> info_v_conv_activated/1
  limit_i_conv*/1 -> Detect Decrease/1, Detect Increase/1
  limit_v_conv*/1 -> Detect Decrease1/1, Detect Increase1/1

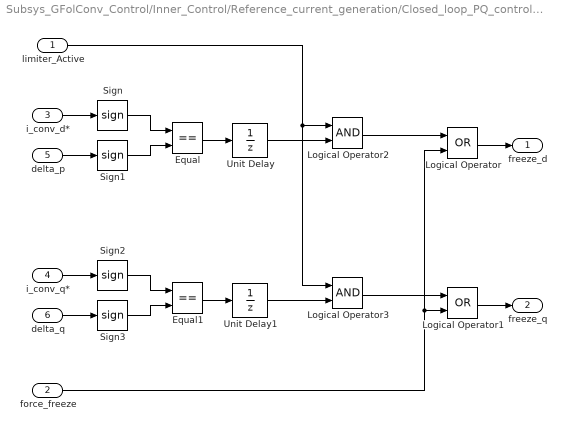
== system Subsys_GFolConv_Control/Inner_Control/Reference_current_generation/Closed_loop_PQ_control/Integrator_Freeze_Logic ==
  limiter_Active : Inport
  force_freeze : Inport  Port=2
  i_conv_d* : Inport  Port=3
  i_conv_q* : Inport  Port=4
  delta_p : Inport  Port=5
  delta_q : Inport  Port=6
  Equal : RelationalOperator  Operator===  OutDataTypeStr=boolean  RndMeth=Simplest  InputSameDT=off
  Equal1 : RelationalOperator  Operator===  OutDataTypeStr=boolean  RndMeth=Simplest  InputSameDT=off
  Logical Operator : Logic  Operator=OR  AllPortsSameDT=off  OutDataTypeStr=boolean
  Logical Operator1 : Logic  Operator=OR  AllPortsSameDT=off  OutDataTypeStr=boolean
  Logical Operator2 : Logic  AllPortsSameDT=off  OutDataTypeStr=boolean
  Logical Operator3 : Logic  AllPortsSameDT=off  OutDataTypeStr=boolean
  Sign{,1..3} (4 alike) : Signum
  Unit Delay : UnitDelay  SampleTime=-1  HasFrameUpgradeWarning=on
  Unit Delay1 : UnitDelay  SampleTime=-1  HasFrameUpgradeWarning=on
  freeze_d : Outport
  freeze_q : Outport  Port=2
  wires:
  Unit Delay1/1 -> Logical Operator3/2
  Unit Delay/1 -> Logical Operator2/2
  i_conv_q*/1 -> Sign2/1
  delta_q/1 -> Sign3/1
  Sign2/1 -> Equal1/1
  Sign3/1 -> Equal1/2
  Equal1/1 -> Unit Delay1/1
  Equal/1 -> Unit Delay/1
  Sign1/1 -> Equal/2
  Sign/1 -> Equal/1
  delta_p/1 -> Sign1/1
  i_conv_d*/1 -> Sign/1
  Logical Operator3/1 -> Logical Operator1/1
  Logical Operator2/1 -> Logical Operator/1
  limiter_Active/1 -> Logical Operator2/1, Logical Operator3/1
  force_freeze/1 -> Logical Operator1/2, Logical Operator/2
  Logical Operator1/1 -> freeze_q/1
  Logical Operator/1 -> freeze_d/1
